simulink model "ElectricVehicleThermalManagementWithHeatPump"  (R2024b)
settings: Solver=VariableStepAuto  StartTime=0.0  StopTime=3600  RelTol=1e-3  AbsTol=1e-3
PreLoadFcn:
  | init_nmpc
InitFcn:
  | init_nmpc
model workspace: external: MATLAB File ElectricVehicleThermalManagementWithHeatPumpParameters.m (data not in the file)
values from neighbouring files (symbols this model uses):
  battery_C1_LUT = [1913.6 12447 30609 ... (first row only)    [ElectricVehicleThermalManagementWithHeatPumpParameters.m]
  battery_capacity_LUT = [280.081 276.25 276.392]    [ElectricVehicleThermalManagementWithHeatPumpParameters.m]
  battery_cell_cp = 795    [ElectricVehicleThermalManagementWithHeatPumpParameters.m]
  battery_cell_mass = 2.5    [ElectricVehicleThermalManagementWithHeatPumpParameters.m]
  battery_Em_LUT = [3.4966 3.5057 3.5148 ... (first row only)    [ElectricVehicleThermalManagementWithHeatPumpParameters.m]
  battery_N_cells = 20    [ElectricVehicleThermalManagementWithHeatPumpParameters.m]
  battery_Qe_init = 0    [ElectricVehicleThermalManagementWithHeatPumpParameters.m]
  battery_R0_LUT = [0.0117 0.0085 0.009 ... (first row only)    [ElectricVehicleThermalManagementWithHeatPumpParameters.m]
  battery_R1_LUT = [0.0109 0.0029 0.0013 ... (first row only)    [ElectricVehicleThermalManagementWithHeatPumpParameters.m]
  battery_SOC_LUT = [0; 0.1; 0.25; 0.5; 0.75; 0.9; 1]    [ElectricVehicleThermalManagementWithHeatPumpParameters.m]
  battery_T_init = -10    [ElectricVehicleThermalManagementWithHeatPumpParameters.m]
  battery_temperature_LUT = [5 20 40]    [ElectricVehicleThermalManagementWithHeatPumpParameters.m]
  cabin_duct_area = 0.04    [ElectricVehicleThermalManagementWithHeatPumpParameters.m]
  cabin_T_init = -10    [ElectricVehicleThermalManagementWithHeatPumpParameters.m]
  chiller_area_primary = 0.43982297150257105    (= 0.439822971503)    [ElectricVehicleThermalManagementWithHeatPumpParameters.m]
  chiller_N_baffles = 3    [ElectricVehicleThermalManagementWithHeatPumpParameters.m]
  chiller_N_tubes = 100    [ElectricVehicleThermalManagementWithHeatPumpParameters.m]
  chiller_tube_D = 0.0035    [ElectricVehicleThermalManagementWithHeatPumpParameters.m]
  chiller_tube_L = 0.4    [ElectricVehicleThermalManagementWithHeatPumpParameters.m]
  chiller_wall_conductivity = 240    [ElectricVehicleThermalManagementWithHeatPumpParameters.m]
  chiller_wall_thickness = 0.0001    [ElectricVehicleThermalManagementWithHeatPumpParameters.m]
  cond_evap_air_area_flow = 0.3906    [ElectricVehicleThermalManagementWithHeatPumpParameters.m]
  cond_evap_air_area_primary = 1.4834999999999998    (= 1.4835)    [ElectricVehicleThermalManagementWithHeatPumpParameters.m]
  cond_evap_W = 0.015    [ElectricVehicleThermalManagementWithHeatPumpParameters.m]
  cond_evap_wall_conductivity = 240    [ElectricVehicleThermalManagementWithHeatPumpParameters.m]
  cond_evap_wall_thickness = 0.0001    [ElectricVehicleThermalManagementWithHeatPumpParameters.m]
  coolant_channel_D = 0.0092    [ElectricVehicleThermalManagementWithHeatPumpParameters.m]
  coolant_pipe_D = 0.019    [ElectricVehicleThermalManagementWithHeatPumpParameters.m]
  coolant_T_init = -10    [ElectricVehicleThermalManagementWithHeatPumpParameters.m]
  coolant_tank_area = 0.0121    [ElectricVehicleThermalManagementWithHeatPumpParameters.m]
  coolant_tank_volume = 1.25    [ElectricVehicleThermalManagementWithHeatPumpParameters.m]
  coolant_valve_D_ratio_max = 0.95    [ElectricVehicleThermalManagementWithHeatPumpParameters.m]
  coolant_valve_D_ratio_min = 0.001    [ElectricVehicleThermalManagementWithHeatPumpParameters.m]
  coolant_valve_displacement = 0.0063    [ElectricVehicleThermalManagementWithHeatPumpParameters.m]
  coolant_valve_S_max = 0.0053    [ElectricVehicleThermalManagementWithHeatPumpParameters.m]
  evaporator_air_area_flow = 0.12    [ElectricVehicleThermalManagementWithHeatPumpParameters.m]
  evaporator_air_area_primary = 0.4323    [ElectricVehicleThermalManagementWithHeatPumpParameters.m]
  evaporator_W = 0.015    [ElectricVehicleThermalManagementWithHeatPumpParameters.m]
  evaporator_wall_conductivity = 240    [ElectricVehicleThermalManagementWithHeatPumpParameters.m]
  evaporator_wall_thickness = 0.0001    [ElectricVehicleThermalManagementWithHeatPumpParameters.m]
  expansion_valve_D_ratio_max = 0.9    [ElectricVehicleThermalManagementWithHeatPumpParameters.m]
  hex_area_primary = 0.070371675440411369    (= 0.0703716754404)    [ElectricVehicleThermalManagementWithHeatPumpParameters.m]
  hex_N_tubes = 64    [ElectricVehicleThermalManagementWithHeatPumpParameters.m]
  hex_tube_D = 0.0035    [ElectricVehicleThermalManagementWithHeatPumpParameters.m]
  hex_wall_conductivity = 240    [ElectricVehicleThermalManagementWithHeatPumpParameters.m]
  hex_wall_thickness = 0.0001    [ElectricVehicleThermalManagementWithHeatPumpParameters.m]
  inner_cond_air_area_flow = 0.1953    [ElectricVehicleThermalManagementWithHeatPumpParameters.m]
  inner_cond_air_area_primary = 0.99520000000000008    (= 0.9952)    [ElectricVehicleThermalManagementWithHeatPumpParameters.m]
  inner_cond_W = 0.02    [ElectricVehicleThermalManagementWithHeatPumpParameters.m]
  inner_cond_wall_conductivity = 240    [ElectricVehicleThermalManagementWithHeatPumpParameters.m]
  inner_cond_wall_thickness = 0.0001    [ElectricVehicleThermalManagementWithHeatPumpParameters.m]
  pump_speed_max = 1000    [ElectricVehicleThermalManagementWithHeatPumpParameters.m]
  radiator_air_area_flow = 0.097499999999999989    (= 0.0975)    [ElectricVehicleThermalManagementWithHeatPumpParameters.m]
  radiator_air_area_primary = 0.43687499999999996    (= 0.436875)    [ElectricVehicleThermalManagementWithHeatPumpParameters.m]
  radiator_W = 0.015    [ElectricVehicleThermalManagementWithHeatPumpParameters.m]
  radiator_wall_conductivity = 240    [ElectricVehicleThermalManagementWithHeatPumpParameters.m]
  radiator_wall_thickness = 0.0001    [ElectricVehicleThermalManagementWithHeatPumpParameters.m]
  refrigerant_p_init = 0.2    [ElectricVehicleThermalManagementWithHeatPumpParameters.m]
  refrigerant_pipe_D = 0.01    [ElectricVehicleThermalManagementWithHeatPumpParameters.m]
  refrigerant_valve_D_ratio_max = 0.95    [ElectricVehicleThermalManagementWithHeatPumpParameters.m]
  refrigerant_valve_displacement = 0.005    [ElectricVehicleThermalManagementWithHeatPumpParameters.m]
libraries: fl_lib x227, nesl_utility x162, SimscapeFluids_lib x30, LiBatteryElements_lib x16, slpidlib x3, SignalEditorBlockLib x1
(part 11 of 13)

== system ElectricVehicleThermalManagementWithHeatPump/Controls/T_battery ==
  MinMax : MinMax  Function=max  Inputs=4
  T_battery : Outport
  wires:
  MinMax/1 -> T_battery/1
  [T_battery1] -> MinMax/1
  [T_battery4] -> MinMax/4
  [T_battery2] -> MinMax/2
  [T_battery3] -> MinMax/3

== system ElectricVehicleThermalManagementWithHeatPump/Controls/Thermal Mode ==
  note: 0 = Off
      |
      | 1 = Cold loop
      |
      | 2 = Heat pump
  T_env : Inport
  rpm_comp : Inport  Port=2
  Mode Selection : Subsystem
  Mode Transition : Subsystem
  Scope : Scope
  To Workspace : ToWorkspace  VariableName=thermal_mode  SampleTime=-1
  thermal_mode : Outport
  wires:
  T_env/1 -> Mode Selection/1(T_env)
  Mode Selection/1(setpoint) -> Scope/1, Mode Transition/1(setpoint)
  Mode Transition/1(thermal_mode) -> To Workspace/1, thermal_mode/1
  rpm_comp/1 -> Mode Transition/2(rpm_comp)

== system ElectricVehicleThermalManagementWithHeatPump/Controls/Valves Control ==
  thermal_mode : Inport
  T_coolant_inverter_out : Inport  Port=2
  T_coolant_battery_in : Inport  Port=3
  T_env : Inport  Port=4
  Chiller Expansion Valve : Subsystem
  Evaporator Expansion Valve : Subsystem
  Heat Pump Expansion Valve : Subsystem
  Radiator 3-Way Valve : Subsystem
  Refrigerant and Air 3-Way Valve : Subsystem
  To Workspace1 : ToWorkspace  VariableName=clntInverterTemp_out  SampleTime=-1
  To Workspace2 : ToWorkspace  VariableName=clntBatTemp_in  SampleTime=-1
  To Workspace3 : ToWorkspace  VariableName=envTemp  SampleTime=-1
  To Workspace4 : ToWorkspace  VariableName=cmdRefByPass  SampleTime=-1
  To Workspace5 : ToWorkspace  VariableName=cmdBlendAir  SampleTime=-1
  To Workspace6 : ToWorkspace  VariableName=cmdRadByPass  SampleTime=-1
  To Workspace7 : ToWorkspace  VariableName=cmdExvChill  SampleTime=-1
  To Workspace8 : ToWorkspace  VariableName=cmdExvEvap  SampleTime=-1
  To Workspace9 : ToWorkspace  VariableName=cmdExvHeatpump  SampleTime=-1
  cmd_refrig_bypass : Outport
  cmd_blend_air : Outport  Port=2
  cmd_rad_bypass : Outport  Port=3
  cmd_exv_chiller : Outport  Port=4
  cmd_exv_evap : Outport  Port=5
  cmd_exv_heatpump : Outport  Port=6
  wires:
  Refrigerant and Air 3-Way Valve/1(cmd_refrig_bypass) -> To Workspace4/1, cmd_refrig_bypass/1
  Refrigerant and Air 3-Way Valve/2(cmd_blend_air) -> To Workspace5/1, cmd_blend_air/1
  T_env/1 -> To Workspace3/1, Heat Pump Expansion Valve/2(T_env), Evaporator Expansion Valve/2(T_env)
  T_coolant_battery_in/1 -> To Workspace2/1, Chiller Expansion Valve/2(T_coolant_battery_in)
  T_coolant_inverter_out/1 -> To Workspace1/1, Radiator 3-Way Valve/2(T_coolant_inverter_out)
  thermal_mode/1 -> Radiator 3-Way Valve/1(thermal_mode), Chiller Expansion Valve/1(thermal_mode), Evaporator Expansion Valve/1(thermal_mode), Heat Pump Expansion Valve/1(thermal_mode), Refrigerant and Air 3-Way Valve/1(thermal_mode)
  Radiator 3-Way Valve/1(cmd_rad_bypass) -> To Workspace6/1, cmd_rad_bypass/1
  Chiller Expansion Valve/1(cmd_exv_chiller) -> To Workspace7/1, cmd_exv_chiller/1
  Evaporator Expansion Valve/1(cmd_exv_evap) -> To Workspace8/1, cmd_exv_evap/1
  Heat Pump Expansion Valve/1(cmd_exv_heatpump) -> To Workspace9/1, cmd_exv_heatpump/1

== system ElectricVehicleThermalManagementWithHeatPump/Evaporator/SR7 ==
  Flow Rate Sensor (2P) : fl_lib/Two-Phase Fluid/Sensors/Flow Rate Sensor (2P)  mass_flow_measure=true  volumetric_flow_measure=false  energy_flow_measure=true
      settings: InternalSimscapePortConfiguration="{\"Bottom\":[{\"id\":\"PHI\",\"label\":\"φ\",\"type\":\"output\"}],\"Left\":[{\"id\":\"A\",\"label\":\"A\",\"type\":\"foundation.two_phase_fluid.two_phase_fluid\"}],\"Right\":[{\"id\":\"B\",\"label\":\"B\",\"type\":\"foundation.two_phase_fluid.two_phase_fluid\"},{\"id\":\"M\",\"label\":\"M\",\"type\":\"output\"}],\"Top\":[]}"
  PS-Simulink Converter : nesl_utility/PS-Simulink Converter  PhysicalDomain=network_engine_domain  SubClassName=ps_output  LeftPortType=input  RightPortType=output  PseudoPeriodic=off  Frequencies=[]  VectorFormat=inherit  Unit=W  AffineConversion=off
  PS-Simulink Converter{1..4} (4 alike) : nesl_utility/PS-Simulink Converter  PhysicalDomain=network_engine_domain  SubClassName=ps_output  LeftPortType=input  RightPortType=output  PseudoPeriodic=off  Frequencies=[]  VectorFormat=inherit  Unit=inherit  AffineConversion=off
  "Pressure, Temperature & Internal Energy Sensor (2P)" : fl_lib/Two-Phase Fluid/Sensors/Pressure, Temperature & Internal Energy Sensor (2P)  reference=foundation.enum.MeasurementReference.absolute  pressure=true  pressure_spec=foundation.enum.PressureMeasementSpec.Absolute  temperature=false  internal_energy=false
      settings: InternalSimscapePortConfiguration="{\"Bottom\":[],\"Left\":[{\"id\":\"A\",\"label\":\"A\",\"type\":\"foundation.two_phase_fluid.two_phase_fluid\"}],\"Right\":[{\"id\":\"Pa\",\"label\":\"Pa\",\"type\":\"output\"}],\"Top\":[]}"
  Thermodynamic Properties Sensor (2P) : fl_lib/Two-Phase Fluid/Sensors/Thermodynamic Properties Sensor (2P)  temperature=true  enthalpy=true  density=true  specific_volume=false  entropy=true
      settings: InternalSimscapePortConfiguration="{\"Bottom\":[{\"id\":\"S\",\"label\":\"s\",\"type\":\"output\"}],\"Left\":[{\"id\":\"A\",\"label\":\"A\",\"type\":\"foundation.two_phase_fluid.two_phase_fluid\"}],\"Right\":[{\"id\":\"T\",\"label\":\"T\",\"type\":\"output\"},{\"id\":\"H\",\"label\":\"h\",\"type\":\"output\"},{\"id\":\"RHO\",\"label\":\"ρ\",\"type\":\"output\"}],\"Top\":[]}"
  To Workspace : ToWorkspace  VariableName=refEvapTemp_in  SampleTime=-1
  To Workspace1 : ToWorkspace  VariableName=refEvapH_in  SampleTime=-1
  To Workspace2 : ToWorkspace  VariableName=refEvapRho_in  SampleTime=-1
  To Workspace3 : ToWorkspace  VariableName=refEvapPres_in  SampleTime=-1
  A : PMIOPort  Side=Left
  B : PMIOPort  Port=2  Side=Right
  tag scope: Phi_evap_in=global
  wires:
  PS-Simulink Converter/1 -> [Phi_evap_in]
  PS-Simulink Converter1/1 -> To Workspace/1
  PS-Simulink Converter2/1 -> To Workspace1/1
  PS-Simulink Converter3/1 -> To Workspace2/1
  PS-Simulink Converter4/1 -> To Workspace3/1
  connections:
  PS-Simulink Converter/LConn1 -- Flow Rate Sensor (2P)/RConn3
  B/RConn1 -- Flow Rate Sensor (2P)/RConn1
  Thermodynamic Properties Sensor (2P)/LConn1 -- A/RConn1 -- "Pressure, Temperature & Internal Energy Sensor (2P)"/LConn1 -- Flow Rate Sensor (2P)/LConn1
  PS-Simulink Converter1/LConn1 -- Thermodynamic Properties Sensor (2P)/RConn1
  PS-Simulink Converter2/LConn1 -- Thermodynamic Properties Sensor (2P)/RConn2
  PS-Simulink Converter3/LConn1 -- Thermodynamic Properties Sensor (2P)/RConn3
  PS-Simulink Converter4/LConn1 -- "Pressure, Temperature & Internal Energy Sensor (2P)"/RConn1

== system ElectricVehicleThermalManagementWithHeatPump/Evaporator/SR8 ==
  Flow Rate Sensor (2P) : fl_lib/Two-Phase Fluid/Sensors/Flow Rate Sensor (2P)  mass_flow_measure=true  volumetric_flow_measure=false  energy_flow_measure=true
      settings: InternalSimscapePortConfiguration="{\"Bottom\":[{\"id\":\"PHI\",\"label\":\"φ\",\"type\":\"output\"}],\"Left\":[{\"id\":\"A\",\"label\":\"A\",\"type\":\"foundation.two_phase_fluid.two_phase_fluid\"}],\"Right\":[{\"id\":\"B\",\"label\":\"B\",\"type\":\"foundation.two_phase_fluid.two_phase_fluid\"},{\"id\":\"M\",\"label\":\"M\",\"type\":\"output\"}],\"Top\":[]}"
  PS-Simulink Converter : nesl_utility/PS-Simulink Converter  PhysicalDomain=network_engine_domain  SubClassName=ps_output  LeftPortType=input  RightPortType=output  PseudoPeriodic=off  Frequencies=[]  VectorFormat=inherit  Unit=W  AffineConversion=off
  PS-Simulink Converter1 : nesl_utility/PS-Simulink Converter  PhysicalDomain=network_engine_domain  SubClassName=ps_output  LeftPortType=input  RightPortType=output  PseudoPeriodic=off  Frequencies=[]  VectorFormat=inherit  Unit=MPa  AffineConversion=off
  PS-Simulink Converter2 : nesl_utility/PS-Simulink Converter  PhysicalDomain=network_engine_domain  SubClassName=ps_output  LeftPortType=input  RightPortType=output  PseudoPeriodic=off  Frequencies=[]  VectorFormat=inherit  Unit=inherit  AffineConversion=off
  PS-Simulink Converter3 : nesl_utility/PS-Simulink Converter  PhysicalDomain=network_engine_domain  SubClassName=ps_output  LeftPortType=input  RightPortType=output  PseudoPeriodic=off  Frequencies=[]  VectorFormat=inherit  Unit=inherit  AffineConversion=off
  PS-Simulink Converter4 : nesl_utility/PS-Simulink Converter  PhysicalDomain=network_engine_domain  SubClassName=ps_output  LeftPortType=input  RightPortType=output  PseudoPeriodic=off  Frequencies=[]  VectorFormat=inherit  Unit=inherit  AffineConversion=off
  "Pressure, Temperature & Internal Energy Sensor (2P)" : fl_lib/Two-Phase Fluid/Sensors/Pressure, Temperature & Internal Energy Sensor (2P)  reference=foundation.enum.MeasurementReference.absolute  pressure=true  pressure_spec=foundation.enum.PressureMeasementSpec.Absolute  temperature=false  internal_energy=false
      settings: InternalSimscapePortConfiguration="{\"Bottom\":[],\"Left\":[{\"id\":\"A\",\"label\":\"A\",\"type\":\"foundation.two_phase_fluid.two_phase_fluid\"}],\"Right\":[{\"id\":\"Pa\",\"label\":\"Pa\",\"type\":\"output\"}],\"Top\":[]}"
  Thermodynamic Properties Sensor (2P) : fl_lib/Two-Phase Fluid/Sensors/Thermodynamic Properties Sensor (2P)  temperature=true  enthalpy=true  density=true  specific_volume=false  entropy=true
      settings: InternalSimscapePortConfiguration="{\"Bottom\":[{\"id\":\"S\",\"label\":\"s\",\"type\":\"output\"}],\"Left\":[{\"id\":\"A\",\"label\":\"A\",\"type\":\"foundation.two_phase_fluid.two_phase_fluid\"}],\"Right\":[{\"id\":\"T\",\"label\":\"T\",\"type\":\"output\"},{\"id\":\"H\",\"label\":\"h\",\"type\":\"output\"},{\"id\":\"RHO\",\"label\":\"ρ\",\"type\":\"output\"}],\"Top\":[]}"
  To Workspace : ToWorkspace  VariableName=refEvapPress_out  SampleTime=-1
  To Workspace1 : ToWorkspace  VariableName=refEvapTemp_out  SampleTime=-1
  To Workspace2 : ToWorkspace  VariableName=refEvapH_out  SampleTime=-1
  To Workspace3 : ToWorkspace  VariableName=refEvapRho_out  SampleTime=-1
  A : PMIOPort  Side=Left
  B : PMIOPort  Port=2  Side=Right
  tag scope: Phi_evap_out=global, p_evap_out=global
  wires:
  PS-Simulink Converter/1 -> [Phi_evap_out]
  PS-Simulink Converter1/1 -> To Workspace/1, [p_evap_out]
  PS-Simulink Converter2/1 -> To Workspace1/1
  PS-Simulink Converter3/1 -> To Workspace2/1
  PS-Simulink Converter4/1 -> To Workspace3/1
  connections:
  PS-Simulink Converter/LConn1 -- Flow Rate Sensor (2P)/RConn3
  B/RConn1 -- Flow Rate Sensor (2P)/RConn1
  Thermodynamic Properties Sensor (2P)/LConn1 -- A/RConn1 -- "Pressure, Temperature & Internal Energy Sensor (2P)"/LConn1 -- Flow Rate Sensor (2P)/LConn1
  PS-Simulink Converter1/LConn1 -- "Pressure, Temperature & Internal Energy Sensor (2P)"/RConn1
  PS-Simulink Converter2/LConn1 -- Thermodynamic Properties Sensor (2P)/RConn1
  PS-Simulink Converter3/LConn1 -- Thermodynamic Properties Sensor (2P)/RConn2
  PS-Simulink Converter4/LConn1 -- Thermodynamic Properties Sensor (2P)/RConn3

== system ElectricVehicleThermalManagementWithHeatPump/Heat Exchanger/SR5 ==
  Flow Rate Sensor (2P) : fl_lib/Two-Phase Fluid/Sensors/Flow Rate Sensor (2P)  mass_flow_measure=true  volumetric_flow_measure=false  energy_flow_measure=true
      settings: InternalSimscapePortConfiguration="{\"Bottom\":[{\"id\":\"PHI\",\"label\":\"φ\",\"type\":\"output\"}],\"Left\":[{\"id\":\"A\",\"label\":\"A\",\"type\":\"foundation.two_phase_fluid.two_phase_fluid\"}],\"Right\":[{\"id\":\"B\",\"label\":\"B\",\"type\":\"foundation.two_phase_fluid.two_phase_fluid\"},{\"id\":\"M\",\"label\":\"M\",\"type\":\"output\"}],\"Top\":[]}"
  PS-Simulink Converter : nesl_utility/PS-Simulink Converter  PhysicalDomain=network_engine_domain  SubClassName=ps_output  LeftPortType=input  RightPortType=output  PseudoPeriodic=off  Frequencies=[]  VectorFormat=inherit  Unit=W  AffineConversion=off
  PS-Simulink Converter1 : nesl_utility/PS-Simulink Converter  PhysicalDomain=network_engine_domain  SubClassName=ps_output  LeftPortType=input  RightPortType=output  PseudoPeriodic=off  Frequencies=[]  VectorFormat=inherit  Unit=inherit  AffineConversion=off
  PS-Simulink Converter2 : nesl_utility/PS-Simulink Converter  PhysicalDomain=network_engine_domain  SubClassName=ps_output  LeftPortType=input  RightPortType=output  PseudoPeriodic=off  Frequencies=[]  VectorFormat=inherit  Unit=inherit  AffineConversion=off
  PS-Simulink Converter3 : nesl_utility/PS-Simulink Converter  PhysicalDomain=network_engine_domain  SubClassName=ps_output  LeftPortType=input  RightPortType=output  PseudoPeriodic=off  Frequencies=[]  VectorFormat=inherit  Unit=inherit  AffineConversion=off
  "Pressure, Temperature & Internal Energy Sensor (2P)" : fl_lib/Two-Phase Fluid/Sensors/Pressure, Temperature & Internal Energy Sensor (2P)  reference=foundation.enum.MeasurementReference.absolute  pressure=true  pressure_spec=foundation.enum.PressureMeasementSpec.Absolute  temperature=false  internal_energy=false
      settings: InternalSimscapePortConfiguration="{\"Bottom\":[],\"Left\":[{\"id\":\"A\",\"label\":\"A\",\"type\":\"foundation.two_phase_fluid.two_phase_fluid\"}],\"Right\":[{\"id\":\"Pa\",\"label\":\"Pa\",\"type\":\"output\"}],\"Top\":[]}"
  Scope : Scope
  Scope1 : Scope
  Scope2 : Scope
  Thermodynamic Properties Sensor (2P) : fl_lib/Two-Phase Fluid/Sensors/Thermodynamic Properties Sensor (2P)  temperature=true  enthalpy=true  density=true  specific_volume=false  entropy=true
      settings: InternalSimscapePortConfiguration="{\"Bottom\":[{\"id\":\"S\",\"label\":\"s\",\"type\":\"output\"}],\"Left\":[{\"id\":\"A\",\"label\":\"A\",\"type\":\"foundation.two_phase_fluid.two_phase_fluid\"}],\"Right\":[{\"id\":\"T\",\"label\":\"T\",\"type\":\"output\"},{\"id\":\"H\",\"label\":\"h\",\"type\":\"output\"},{\"id\":\"RHO\",\"label\":\"ρ\",\"type\":\"output\"}],\"Top\":[]}"
  To Workspace : ToWorkspace  VariableName=heatExchangerRefPress_inPa  SampleTime=-1
  To Workspace1 : ToWorkspace  VariableName=heatExchangerRefTemp_inK  SampleTime=-1
  To Workspace2 : ToWorkspace  VariableName=heatExchangerRefEnthaply_in  SampleTime=-1
  A : PMIOPort  Side=Left
  B : PMIOPort  Port=2  Side=Right
  tag scope: Phi_hex_in=global
  wires:
  PS-Simulink Converter/1 -> [Phi_hex_in]
  PS-Simulink Converter2/1 -> Scope/1, To Workspace/1
  PS-Simulink Converter1/1 -> Scope1/1, To Workspace1/1
  PS-Simulink Converter3/1 -> Scope2/1, To Workspace2/1
  connections:
  PS-Simulink Converter/LConn1 -- Flow Rate Sensor (2P)/RConn3
  B/RConn1 -- Flow Rate Sensor (2P)/RConn1
  Thermodynamic Properties Sensor (2P)/LConn1 -- A/RConn1 -- "Pressure, Temperature & Internal Energy Sensor (2P)"/LConn1 -- Flow Rate Sensor (2P)/LConn1
  PS-Simulink Converter1/LConn1 -- Thermodynamic Properties Sensor (2P)/RConn1
  PS-Simulink Converter2/LConn1 -- "Pressure, Temperature & Internal Energy Sensor (2P)"/RConn1
  Thermodynamic Properties Sensor (2P)/RConn2 -- PS-Simulink Converter3/LConn1

== system ElectricVehicleThermalManagementWithHeatPump/Heat Exchanger/SR6 ==
  Flow Rate Sensor (2P) : fl_lib/Two-Phase Fluid/Sensors/Flow Rate Sensor (2P)  mass_flow_measure=true  volumetric_flow_measure=false  energy_flow_measure=true
      settings: InternalSimscapePortConfiguration="{\"Bottom\":[{\"id\":\"PHI\",\"label\":\"φ\",\"type\":\"output\"}],\"Left\":[{\"id\":\"A\",\"label\":\"A\",\"type\":\"foundation.two_phase_fluid.two_phase_fluid\"}],\"Right\":[{\"id\":\"B\",\"label\":\"B\",\"type\":\"foundation.two_phase_fluid.two_phase_fluid\"},{\"id\":\"M\",\"label\":\"M\",\"type\":\"output\"}],\"Top\":[]}"
  PS-Simulink Converter : nesl_utility/PS-Simulink Converter  PhysicalDomain=network_engine_domain  SubClassName=ps_output  LeftPortType=input  RightPortType=output  PseudoPeriodic=off  Frequencies=[]  VectorFormat=inherit  Unit=W  AffineConversion=off
  PS-Simulink Converter1 : nesl_utility/PS-Simulink Converter  PhysicalDomain=network_engine_domain  SubClassName=ps_output  LeftPortType=input  RightPortType=output  PseudoPeriodic=off  Frequencies=[]  VectorFormat=inherit  Unit=inherit  AffineConversion=off
  PS-Simulink Converter2 : nesl_utility/PS-Simulink Converter  PhysicalDomain=network_engine_domain  SubClassName=ps_output  LeftPortType=input  RightPortType=output  PseudoPeriodic=off  Frequencies=[]  VectorFormat=inherit  Unit=inherit  AffineConversion=off
  PS-Simulink Converter3 : nesl_utility/PS-Simulink Converter  PhysicalDomain=network_engine_domain  SubClassName=ps_output  LeftPortType=input  RightPortType=output  PseudoPeriodic=off  Frequencies=[]  VectorFormat=inherit  Unit=inherit  AffineConversion=off
  "Pressure, Temperature & Internal Energy Sensor (2P)" : fl_lib/Two-Phase Fluid/Sensors/Pressure, Temperature & Internal Energy Sensor (2P)  reference=foundation.enum.MeasurementReference.absolute  pressure=true  pressure_spec=foundation.enum.PressureMeasementSpec.Absolute  temperature=false  internal_energy=false
      settings: InternalSimscapePortConfiguration="{\"Bottom\":[],\"Left\":[{\"id\":\"A\",\"label\":\"A\",\"type\":\"foundation.two_phase_fluid.two_phase_fluid\"}],\"Right\":[{\"id\":\"Pa\",\"label\":\"Pa\",\"type\":\"output\"}],\"Top\":[]}"
  Scope : Scope
  Scope1 : Scope
  Scope2 : Scope
  Thermodynamic Properties Sensor (2P) : fl_lib/Two-Phase Fluid/Sensors/Thermodynamic Properties Sensor (2P)  temperature=true  enthalpy=true  density=true  specific_volume=false  entropy=true
      settings: InternalSimscapePortConfiguration="{\"Bottom\":[{\"id\":\"S\",\"label\":\"s\",\"type\":\"output\"}],\"Left\":[{\"id\":\"A\",\"label\":\"A\",\"type\":\"foundation.two_phase_fluid.two_phase_fluid\"}],\"Right\":[{\"id\":\"T\",\"label\":\"T\",\"type\":\"output\"},{\"id\":\"H\",\"label\":\"h\",\"type\":\"output\"},{\"id\":\"RHO\",\"label\":\"ρ\",\"type\":\"output\"}],\"Top\":[]}"
  To Workspace : ToWorkspace  VariableName=heatExchangerRefPress_outPa  SampleTime=-1
  To Workspace1 : ToWorkspace  VariableName=heatExchangerRefTemp_outK  SampleTime=-1
  To Workspace2 : ToWorkspace  VariableName=heatExchangerRefEnthaply_out  SampleTime=-1
  A : PMIOPort  Side=Left
  B : PMIOPort  Port=2  Side=Right
  tag scope: Phi_hex_out=global
  wires:
  PS-Simulink Converter/1 -> [Phi_hex_out]
  PS-Simulink Converter1/1 -> Scope/1, To Workspace/1
  PS-Simulink Converter2/1 -> Scope1/1, To Workspace1/1
  PS-Simulink Converter3/1 -> Scope2/1, To Workspace2/1
  connections:
  PS-Simulink Converter/LConn1 -- Flow Rate Sensor (2P)/RConn3
  B/RConn1 -- Flow Rate Sensor (2P)/RConn1
  Thermodynamic Properties Sensor (2P)/LConn1 -- A/RConn1 -- "Pressure, Temperature & Internal Energy Sensor (2P)"/LConn1 -- Flow Rate Sensor (2P)/LConn1
  PS-Simulink Converter1/LConn1 -- "Pressure, Temperature & Internal Energy Sensor (2P)"/RConn1
  PS-Simulink Converter2/LConn1 -- Thermodynamic Properties Sensor (2P)/RConn1
  PS-Simulink Converter3/LConn1 -- Thermodynamic Properties Sensor (2P)/RConn2

== system ElectricVehicleThermalManagementWithHeatPump/Inner Condenser/SR1 ==
  Flow Rate Sensor (2P) : fl_lib/Two-Phase Fluid/Sensors/Flow Rate Sensor (2P)  mass_flow_measure=true  volumetric_flow_measure=false  energy_flow_measure=true
      settings: InternalSimscapePortConfiguration="{\"Bottom\":[{\"id\":\"PHI\",\"label\":\"φ\",\"type\":\"output\"}],\"Left\":[{\"id\":\"A\",\"label\":\"A\",\"type\":\"foundation.two_phase_fluid.two_phase_fluid\"}],\"Right\":[{\"id\":\"B\",\"label\":\"B\",\"type\":\"foundation.two_phase_fluid.two_phase_fluid\"},{\"id\":\"M\",\"label\":\"M\",\"type\":\"output\"}],\"Top\":[]}"
  PS-Simulink Converter : nesl_utility/PS-Simulink Converter  PhysicalDomain=network_engine_domain  SubClassName=ps_output  LeftPortType=input  RightPortType=output  PseudoPeriodic=off  Frequencies=[]  VectorFormat=inherit  Unit=W  AffineConversion=off
  PS-Simulink Converter{1..4} (4 alike) : nesl_utility/PS-Simulink Converter  PhysicalDomain=network_engine_domain  SubClassName=ps_output  LeftPortType=input  RightPortType=output  PseudoPeriodic=off  Frequencies=[]  VectorFormat=inherit  Unit=inherit  AffineConversion=off
  "Pressure, Temperature & Internal Energy Sensor (2P)" : fl_lib/Two-Phase Fluid/Sensors/Pressure, Temperature & Internal Energy Sensor (2P)  reference=foundation.enum.MeasurementReference.absolute  pressure=true  pressure_spec=foundation.enum.PressureMeasementSpec.Absolute  temperature=false  internal_energy=false
      settings: InternalSimscapePortConfiguration="{\"Bottom\":[],\"Left\":[{\"id\":\"A\",\"label\":\"A\",\"type\":\"foundation.two_phase_fluid.two_phase_fluid\"}],\"Right\":[{\"id\":\"Pa\",\"label\":\"Pa\",\"type\":\"output\"}],\"Top\":[]}"
  Scope{,1..3} (4 alike) : Scope
  Thermodynamic Properties Sensor (2P) : fl_lib/Two-Phase Fluid/Sensors/Thermodynamic Properties Sensor (2P)  temperature=true  enthalpy=true  density=true  specific_volume=false  entropy=true
      settings: InternalSimscapePortConfiguration="{\"Bottom\":[{\"id\":\"S\",\"label\":\"s\",\"type\":\"output\"}],\"Left\":[{\"id\":\"A\",\"label\":\"A\",\"type\":\"foundation.two_phase_fluid.two_phase_fluid\"}],\"Right\":[{\"id\":\"T\",\"label\":\"T\",\"type\":\"output\"},{\"id\":\"H\",\"label\":\"h\",\"type\":\"output\"},{\"id\":\"RHO\",\"label\":\"ρ\",\"type\":\"output\"}],\"Top\":[]}"
  To Workspace : ToWorkspace  VariableName=innerCondRefPress_inMPa  SampleTime=-1
  To Workspace1 : ToWorkspace  VariableName=RefMassFlowRate  SampleTime=-1
  To Workspace2 : ToWorkspace  VariableName=innerCondRefTemp_inK  SampleTime=-1
  To Workspace3 : ToWorkspace  VariableName=innerCondRefEnthaply_in  SampleTime=-1
  A : PMIOPort  Side=Left
  B : PMIOPort  Port=2  Side=Right
  tag scope: Phi_inner_cond_in=global
  wires:
  PS-Simulink Converter/1 -> [Phi_inner_cond_in]
  PS-Simulink Converter1/1 -> Scope/1, To Workspace/1
  PS-Simulink Converter2/1 -> Scope1/1, To Workspace1/1
  PS-Simulink Converter3/1 -> Scope2/1, To Workspace2/1
  PS-Simulink Converter4/1 -> Scope3/1, To Workspace3/1
  connections:
  PS-Simulink Converter/LConn1 -- Flow Rate Sensor (2P)/RConn3
  B/RConn1 -- Flow Rate Sensor (2P)/RConn1
  Thermodynamic Properties Sensor (2P)/LConn1 -- A/RConn1 -- "Pressure, Temperature & Internal Energy Sensor (2P)"/LConn1 -- Flow Rate Sensor (2P)/LConn1
  PS-Simulink Converter1/LConn1 -- "Pressure, Temperature & Internal Energy Sensor (2P)"/RConn1
  PS-Simulink Converter2/LConn1 -- Flow Rate Sensor (2P)/RConn2
  PS-Simulink Converter3/LConn1 -- Thermodynamic Properties Sensor (2P)/RConn1
  PS-Simulink Converter4/LConn1 -- Thermodynamic Properties Sensor (2P)/RConn2

== system ElectricVehicleThermalManagementWithHeatPump/Inner Condenser/SR2 ==
  Flow Rate Sensor (2P) : fl_lib/Two-Phase Fluid/Sensors/Flow Rate Sensor (2P)  mass_flow_measure=true  volumetric_flow_measure=false  energy_flow_measure=true
      settings: InternalSimscapePortConfiguration="{\"Bottom\":[{\"id\":\"PHI\",\"label\":\"φ\",\"type\":\"output\"}],\"Left\":[{\"id\":\"A\",\"label\":\"A\",\"type\":\"foundation.two_phase_fluid.two_phase_fluid\"}],\"Right\":[{\"id\":\"B\",\"label\":\"B\",\"type\":\"foundation.two_phase_fluid.two_phase_fluid\"},{\"id\":\"M\",\"label\":\"M\",\"type\":\"output\"}],\"Top\":[]}"
  PS-Simulink Converter : nesl_utility/PS-Simulink Converter  PhysicalDomain=network_engine_domain  SubClassName=ps_output  LeftPortType=input  RightPortType=output  PseudoPeriodic=off  Frequencies=[]  VectorFormat=inherit  Unit=W  AffineConversion=off
  PS-Simulink Converter1 : nesl_utility/PS-Simulink Converter  PhysicalDomain=network_engine_domain  SubClassName=ps_output  LeftPortType=input  RightPortType=output  PseudoPeriodic=off  Frequencies=[]  VectorFormat=inherit  Unit=MPa  AffineConversion=off
  PS-Simulink Converter2 : nesl_utility/PS-Simulink Converter  PhysicalDomain=network_engine_domain  SubClassName=ps_output  LeftPortType=input  RightPortType=output  PseudoPeriodic=off  Frequencies=[]  VectorFormat=inherit  Unit=inherit  AffineConversion=off
  PS-Simulink Converter3 : nesl_utility/PS-Simulink Converter  PhysicalDomain=network_engine_domain  SubClassName=ps_output  LeftPortType=input  RightPortType=output  PseudoPeriodic=off  Frequencies=[]  VectorFormat=inherit  Unit=inherit  AffineConversion=off
  "Pressure, Temperature & Internal Energy Sensor (2P)" : fl_lib/Two-Phase Fluid/Sensors/Pressure, Temperature & Internal Energy Sensor (2P)  reference=foundation.enum.MeasurementReference.absolute  pressure=true  pressure_spec=foundation.enum.PressureMeasementSpec.Absolute  temperature=false  internal_energy=false
      settings: InternalSimscapePortConfiguration="{\"Bottom\":[],\"Left\":[{\"id\":\"A\",\"label\":\"A\",\"type\":\"foundation.two_phase_fluid.two_phase_fluid\"}],\"Right\":[{\"id\":\"Pa\",\"label\":\"Pa\",\"type\":\"output\"}],\"Top\":[]}"
  Thermodynamic Properties Sensor (2P) : fl_lib/Two-Phase Fluid/Sensors/Thermodynamic Properties Sensor (2P)  temperature=true  enthalpy=true  density=true  specific_volume=false  entropy=true
      settings: InternalSimscapePortConfiguration="{\"Bottom\":[{\"id\":\"S\",\"label\":\"s\",\"type\":\"output\"}],\"Left\":[{\"id\":\"A\",\"label\":\"A\",\"type\":\"foundation.two_phase_fluid.two_phase_fluid\"}],\"Right\":[{\"id\":\"T\",\"label\":\"T\",\"type\":\"output\"},{\"id\":\"H\",\"label\":\"h\",\"type\":\"output\"},{\"id\":\"RHO\",\"label\":\"ρ\",\"type\":\"output\"}],\"Top\":[]}"
  To Workspace : ToWorkspace  VariableName=innerCondRefPress_outMpa  SampleTime=-1
  To Workspace1 : ToWorkspace  VariableName=innerCondRefTemp_outK  SampleTime=-1
  To Workspace2 : ToWorkspace  VariableName=innerCondRefEnthaply_out  SampleTime=-1
  A : PMIOPort  Side=Left
  B : PMIOPort  Port=2  Side=Right
  tag scope: Phi_inner_cond_out=global, p_inner_cond_out=global
  wires:
  PS-Simulink Converter/1 -> [Phi_inner_cond_out]
  PS-Simulink Converter1/1 -> To Workspace/1, [p_inner_cond_out]
  PS-Simulink Converter2/1 -> To Workspace1/1
  PS-Simulink Converter3/1 -> To Workspace2/1
  connections:
  PS-Simulink Converter/LConn1 -- Flow Rate Sensor (2P)/RConn3
  B/RConn1 -- Flow Rate Sensor (2P)/RConn1
  Thermodynamic Properties Sensor (2P)/LConn1 -- A/RConn1 -- "Pressure, Temperature & Internal Energy Sensor (2P)"/LConn1 -- Flow Rate Sensor (2P)/LConn1
  PS-Simulink Converter1/LConn1 -- "Pressure, Temperature & Internal Energy Sensor (2P)"/RConn1
  PS-Simulink Converter2/LConn1 -- Thermodynamic Properties Sensor (2P)/RConn1
  PS-Simulink Converter3/LConn1 -- Thermodynamic Properties Sensor (2P)/RConn2

== system ElectricVehicleThermalManagementWithHeatPump/Inverter/SC7 ==
  Flow Rate Sensor (TL) : fl_lib/Thermal Liquid/Sensors/Flow Rate Sensor (TL)  mass_flow_measure=true  volumetric_flow_measure=false  energy_flow_measure=true
      settings: InternalSimscapePortConfiguration="{\"Bottom\":[{\"id\":\"PHI\",\"label\":\"φ\",\"type\":\"output\"}],\"Left\":[{\"id\":\"A\",\"label\":\"A\",\"type\":\"foundation.thermal_liquid.thermal_liquid\"}],\"Right\":[{\"id\":\"B\",\"label\":\"B\",\"type\":\"foundation.thermal_liquid.thermal_liquid\"},{\"id\":\"M\",\"label\":\"M\",\"type\":\"output\"}],\"Top\":[]}"
  PS-Simulink Converter1 : nesl_utility/PS-Simulink Converter  PhysicalDomain=network_engine_domain  SubClassName=ps_output  LeftPortType=input  RightPortType=output  PseudoPeriodic=off  Frequencies=[]  VectorFormat=inherit  Unit=degC  AffineConversion=on
  Pressure & Temperature Sensor (TL) : fl_lib/Thermal Liquid/Sensors/Pressure & Temperature Sensor (TL)  reference=foundation.enum.MeasurementReference.absolute  pressure=true  pressure_spec=foundation.enum.PressureMeasementSpec.Absolute  temperature=true
      settings: InternalSimscapePortConfiguration="{\"Bottom\":[{\"id\":\"T\",\"label\":\"T\",\"type\":\"output\"}],\"Left\":[{\"id\":\"A\",\"label\":\"A\",\"type\":\"foundation.thermal_liquid.thermal_liquid\"}],\"Right\":[{\"id\":\"Pa\",\"label\":\"Pa\",\"type\":\"output\"}],\"Top\":[]}"
  A : PMIOPort  Side=Left
  B : PMIOPort  Port=2  Side=Right
  tag scope: T_coolant_inverter_out=global
  wires:
  PS-Simulink Converter1/1 -> [T_coolant_inverter_out]
  connections:
  B/RConn1 -- Flow Rate Sensor (TL)/RConn1
  Flow Rate Sensor (TL)/LConn1 -- Pressure & Temperature Sensor (TL)/LConn1 -- A/RConn1
  PS-Simulink Converter1/LConn1 -- Pressure & Temperature Sensor (TL)/RConn2

== system ElectricVehicleThermalManagementWithHeatPump/Motor/SC5 ==
  Flow Rate Sensor (TL) : fl_lib/Thermal Liquid/Sensors/Flow Rate Sensor (TL)  mass_flow_measure=true  volumetric_flow_measure=false  energy_flow_measure=true
      settings: InternalSimscapePortConfiguration="{\"Bottom\":[{\"id\":\"PHI\",\"label\":\"φ\",\"type\":\"output\"}],\"Left\":[{\"id\":\"A\",\"label\":\"A\",\"type\":\"foundation.thermal_liquid.thermal_liquid\"}],\"Right\":[{\"id\":\"B\",\"label\":\"B\",\"type\":\"foundation.thermal_liquid.thermal_liquid\"},{\"id\":\"M\",\"label\":\"M\",\"type\":\"output\"}],\"Top\":[]}"
  PS-Simulink Converter : nesl_utility/PS-Simulink Converter  PhysicalDomain=network_engine_domain  SubClassName=ps_output  LeftPortType=input  RightPortType=output  PseudoPeriodic=off  Frequencies=[]  VectorFormat=inherit  Unit=W  AffineConversion=off
  Pressure & Temperature Sensor (TL) : fl_lib/Thermal Liquid/Sensors/Pressure & Temperature Sensor (TL)  reference=foundation.enum.MeasurementReference.absolute  pressure=true  pressure_spec=foundation.enum.PressureMeasementSpec.Absolute  temperature=true
      settings: InternalSimscapePortConfiguration="{\"Bottom\":[{\"id\":\"T\",\"label\":\"T\",\"type\":\"output\"}],\"Left\":[{\"id\":\"A\",\"label\":\"A\",\"type\":\"foundation.thermal_liquid.thermal_liquid\"}],\"Right\":[{\"id\":\"Pa\",\"label\":\"Pa\",\"type\":\"output\"}],\"Top\":[]}"
  A : PMIOPort  Side=Left
  B : PMIOPort  Port=2  Side=Right
  tag scope: Phi_motor_in=global
  wires:
  PS-Simulink Converter/1 -> [Phi_motor_in]
  connections:
  B/RConn1 -- Flow Rate Sensor (TL)/RConn1
  Flow Rate Sensor (TL)/LConn1 -- Pressure & Temperature Sensor (TL)/LConn1 -- A/RConn1
  PS-Simulink Converter/LConn1 -- Flow Rate Sensor (TL)/RConn3

== system ElectricVehicleThermalManagementWithHeatPump/Motor/SC6 ==
  Flow Rate Sensor (TL) : fl_lib/Thermal Liquid/Sensors/Flow Rate Sensor (TL)  mass_flow_measure=true  volumetric_flow_measure=false  energy_flow_measure=true
      settings: InternalSimscapePortConfiguration="{\"Bottom\":[{\"id\":\"PHI\",\"label\":\"φ\",\"type\":\"output\"}],\"Left\":[{\"id\":\"A\",\"label\":\"A\",\"type\":\"foundation.thermal_liquid.thermal_liquid\"}],\"Right\":[{\"id\":\"B\",\"label\":\"B\",\"type\":\"foundation.thermal_liquid.thermal_liquid\"},{\"id\":\"M\",\"label\":\"M\",\"type\":\"output\"}],\"Top\":[]}"
  PS-Simulink Converter : nesl_utility/PS-Simulink Converter  PhysicalDomain=network_engine_domain  SubClassName=ps_output  LeftPortType=input  RightPortType=output  PseudoPeriodic=off  Frequencies=[]  VectorFormat=inherit  Unit=W  AffineConversion=off
  Pressure & Temperature Sensor (TL) : fl_lib/Thermal Liquid/Sensors/Pressure & Temperature Sensor (TL)  reference=foundation.enum.MeasurementReference.absolute  pressure=true  pressure_spec=foundation.enum.PressureMeasementSpec.Absolute  temperature=true
      settings: InternalSimscapePortConfiguration="{\"Bottom\":[{\"id\":\"T\",\"label\":\"T\",\"type\":\"output\"}],\"Left\":[{\"id\":\"A\",\"label\":\"A\",\"type\":\"foundation.thermal_liquid.thermal_liquid\"}],\"Right\":[{\"id\":\"Pa\",\"label\":\"Pa\",\"type\":\"output\"}],\"Top\":[]}"
  A : PMIOPort  Side=Left
  B : PMIOPort  Port=2  Side=Right
  tag scope: Phi_motor_out=global
  wires:
  PS-Simulink Converter/1 -> [Phi_motor_out]
  connections:
  B/RConn1 -- Flow Rate Sensor (TL)/RConn1
  Flow Rate Sensor (TL)/LConn1 -- Pressure & Temperature Sensor (TL)/LConn1 -- A/RConn1
  PS-Simulink Converter/LConn1 -- Flow Rate Sensor (TL)/RConn3

== system ElectricVehicleThermalManagementWithHeatPump/Motor Pump/Heat Transfer ==
  Convective Heat Transfer : fl_lib/Thermal/Thermal Elements/Convective Heat Transfer  thermal_type=foundation.enum.constant_variable.constant  area=3 * coolant_tank_area m^2  heat_tr_coeff=20 W/(m^2 * K)  min_heat_tr_coeff=1e-3 W/(K*m^2)  T_specify=off  T_priority=None  T=0 K  T_nominal_specify=off  T_nominal_value=1  T_nominal_unit=K  Q_specify=off  Q_priority=None  Q=0 W  Q_nominal_specify=off  Q_nominal_value=1  Q_nominal_unit=W
  Convective Heat Transfer1 : fl_lib/Thermal/Thermal Elements/Convective Heat Transfer  thermal_type=foundation.enum.constant_variable.constant  area=3 * coolant_tank_area m^2  heat_tr_coeff=20 W/(m^2 * K)  min_heat_tr_coeff=1e-3 W/(K*m^2)  T_specify=off  T_priority=None  T=0 K  T_nominal_specify=off  T_nominal_value=1  T_nominal_unit=K  Q_specify=off  Q_priority=None  Q=0 W  Q_nominal_specify=off  Q_nominal_value=1  Q_nominal_unit=W
  Environment Temperature : fl_lib/Thermal/Thermal Sources/Controlled Temperature Source
  Simulink-PS Converter : nesl_utility/Simulink-PS Converter  PhysicalDomain=network_engine_domain  SubClassName=ps_input  LeftPortType=input  RightPortType=output  PseudoPeriodic=off  Frequencies=[]  NoiseDistribution=none  NoiseParameters=[]  Unit=degC  AffineConversion=on  FilteringAndDerivatives=provide  SimscapeFilterOrder=1  InputFilterTimeConstant=0.001  UdotUserProvided=0
  Thermal Reference : fl_lib/Thermal/Thermal Elements/Thermal Reference
  A : PMIOPort  Side=Right
  B : PMIOPort  Port=2  Side=Right
  wires:
  [T_env] -> Simulink-PS Converter/1
  connections:
  Simulink-PS Converter/RConn1 -- Environment Temperature/RConn1
  Thermal Reference/LConn1 -- Environment Temperature/RConn2
  Convective Heat Transfer/RConn1 -- Environment Temperature/LConn1 -- Convective Heat Transfer1/RConn1
  B/RConn1 -- Convective Heat Transfer1/LConn1
  A/RConn1 -- Convective Heat Transfer/LConn1

== system ElectricVehicleThermalManagementWithHeatPump/Radiator/SC1 ==
  Flow Rate Sensor (TL) : fl_lib/Thermal Liquid/Sensors/Flow Rate Sensor (TL)  mass_flow_measure=true  volumetric_flow_measure=false  energy_flow_measure=true
      settings: InternalSimscapePortConfiguration="{\"Bottom\":[{\"id\":\"PHI\",\"label\":\"φ\",\"type\":\"output\"}],\"Left\":[{\"id\":\"A\",\"label\":\"A\",\"type\":\"foundation.thermal_liquid.thermal_liquid\"}],\"Right\":[{\"id\":\"B\",\"label\":\"B\",\"type\":\"foundation.thermal_liquid.thermal_liquid\"},{\"id\":\"M\",\"label\":\"M\",\"type\":\"output\"}],\"Top\":[]}"
  PS-Simulink Converter : nesl_utility/PS-Simulink Converter  PhysicalDomain=network_engine_domain  SubClassName=ps_output  LeftPortType=input  RightPortType=output  PseudoPeriodic=off  Frequencies=[]  VectorFormat=inherit  Unit=W  AffineConversion=off
  PS-Simulink Converter1 : nesl_utility/PS-Simulink Converter  PhysicalDomain=network_engine_domain  SubClassName=ps_output  LeftPortType=input  RightPortType=output  PseudoPeriodic=off  Frequencies=[]  VectorFormat=inherit  Unit=inherit  AffineConversion=off
  Pressure & Temperature Sensor (TL) : fl_lib/Thermal Liquid/Sensors/Pressure & Temperature Sensor (TL)  reference=foundation.enum.MeasurementReference.absolute  pressure=true  pressure_spec=foundation.enum.PressureMeasementSpec.Absolute  temperature=true
      settings: InternalSimscapePortConfiguration="{\"Bottom\":[{\"id\":\"T\",\"label\":\"T\",\"type\":\"output\"}],\"Left\":[{\"id\":\"A\",\"label\":\"A\",\"type\":\"foundation.thermal_liquid.thermal_liquid\"}],\"Right\":[{\"id\":\"Pa\",\"label\":\"Pa\",\"type\":\"output\"}],\"Top\":[]}"
  To Workspace : ToWorkspace  VariableName=clntRadTemp_in  SampleTime=-1
  A : PMIOPort  Side=Left
  B : PMIOPort  Port=2  Side=Right
  tag scope: Phi_rad_in=global
  wires:
  PS-Simulink Converter/1 -> [Phi_rad_in]
  PS-Simulink Converter1/1 -> To Workspace/1
  connections:
  PS-Simulink Converter/LConn1 -- Flow Rate Sensor (TL)/RConn3
  A/RConn1 -- Pressure & Temperature Sensor (TL)/LConn1 -- Flow Rate Sensor (TL)/LConn1
  B/RConn1 -- Flow Rate Sensor (TL)/RConn1
  PS-Simulink Converter1/LConn1 -- Pressure & Temperature Sensor (TL)/RConn2

== system ElectricVehicleThermalManagementWithHeatPump/Radiator/SC2 ==
  Flow Rate Sensor (TL) : fl_lib/Thermal Liquid/Sensors/Flow Rate Sensor (TL)  mass_flow_measure=true  volumetric_flow_measure=false  energy_flow_measure=true
      settings: InternalSimscapePortConfiguration="{\"Bottom\":[{\"id\":\"PHI\",\"label\":\"φ\",\"type\":\"output\"}],\"Left\":[{\"id\":\"A\",\"label\":\"A\",\"type\":\"foundation.thermal_liquid.thermal_liquid\"}],\"Right\":[{\"id\":\"B\",\"label\":\"B\",\"type\":\"foundation.thermal_liquid.thermal_liquid\"},{\"id\":\"M\",\"label\":\"M\",\"type\":\"output\"}],\"Top\":[]}"
  PS-Simulink Converter : nesl_utility/PS-Simulink Converter  PhysicalDomain=network_engine_domain  SubClassName=ps_output  LeftPortType=input  RightPortType=output  PseudoPeriodic=off  Frequencies=[]  VectorFormat=inherit  Unit=W  AffineConversion=off
  PS-Simulink Converter1 : nesl_utility/PS-Simulink Converter  PhysicalDomain=network_engine_domain  SubClassName=ps_output  LeftPortType=input  RightPortType=output  PseudoPeriodic=off  Frequencies=[]  VectorFormat=inherit  Unit=kg/s  AffineConversion=off
  PS-Simulink Converter2 : nesl_utility/PS-Simulink Converter  PhysicalDomain=network_engine_domain  SubClassName=ps_output  LeftPortType=input  RightPortType=output  PseudoPeriodic=off  Frequencies=[]  VectorFormat=inherit  Unit=inherit  AffineConversion=off
  Pressure & Temperature Sensor (TL) : fl_lib/Thermal Liquid/Sensors/Pressure & Temperature Sensor (TL)  reference=foundation.enum.MeasurementReference.absolute  pressure=true  pressure_spec=foundation.enum.PressureMeasementSpec.Absolute  temperature=true
      settings: InternalSimscapePortConfiguration="{\"Bottom\":[{\"id\":\"T\",\"label\":\"T\",\"type\":\"output\"}],\"Left\":[{\"id\":\"A\",\"label\":\"A\",\"type\":\"foundation.thermal_liquid.thermal_liquid\"}],\"Right\":[{\"id\":\"Pa\",\"label\":\"Pa\",\"type\":\"output\"}],\"Top\":[]}"
  Scope : Scope
  To Workspace : ToWorkspace  VariableName=clntRadTemp_out  SampleTime=-1
  A : PMIOPort  Side=Left
  B : PMIOPort  Port=2  Side=Right
  tag scope: Phi_rad_out=global
  wires:
  PS-Simulink Converter/1 -> [Phi_rad_out]
  PS-Simulink Converter1/1 -> Scope/1
  PS-Simulink Converter2/1 -> To Workspace/1
  connections:
  PS-Simulink Converter/LConn1 -- Flow Rate Sensor (TL)/RConn3
  A/RConn1 -- Pressure & Temperature Sensor (TL)/LConn1 -- Flow Rate Sensor (TL)/LConn1
  B/RConn1 -- Flow Rate Sensor (TL)/RConn1
  PS-Simulink Converter1/LConn1 -- Flow Rate Sensor (TL)/RConn2
  PS-Simulink Converter2/LConn1 -- Pressure & Temperature Sensor (TL)/RConn2
